simulink model "srmc_sensor_controller_model"  (R2025a)
settings: Solver=FixedStepDiscrete  StartTime=0.0  StopTime=86400  FixedStep=300  RelTol=1e-3
settings Model: Creator=ELCOT  LastModifiedBy=ELCOT

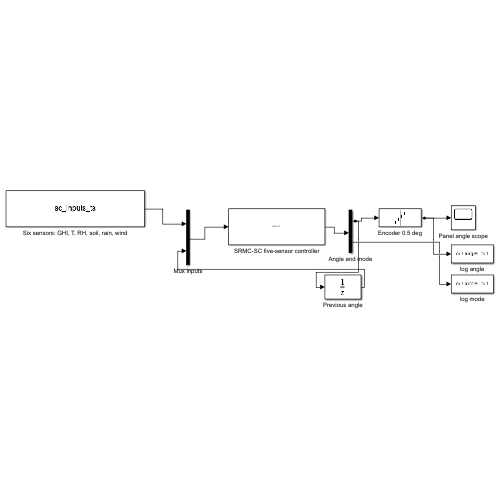
[thumbnail: Simulink's stored preview of the top-level diagram]
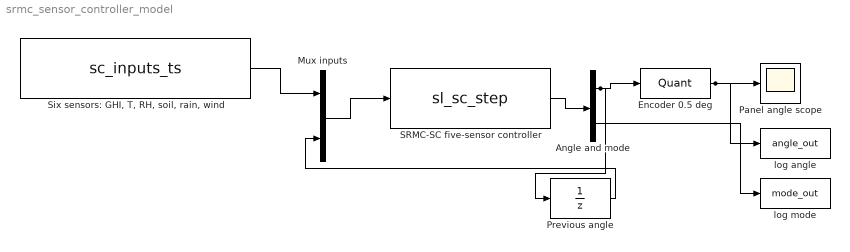
== system srmc_sensor_controller_model ==
  Angle and mode : Demux  Outputs=2
  Encoder 0.5 deg : Quantizer
  Mux inputs : Mux  Inputs=2
  Panel angle scope : Scope
  Previous angle : UnitDelay  InitialCondition=15  SampleTime=300  HasFrameUpgradeWarning=on
  SRMC-SC five-sensor controller : MATLABFcn  MATLABFcn=sl_sc_step  OutputDimensions=2
  "Six sensors: GHI, T, RH, soil, rain, wind" : FromWorkspace  VariableName=sc_inputs_ts  SampleTime=300
  log angle : ToWorkspace  VariableName=angle_out  SampleTime=-1
  log mode : ToWorkspace  VariableName=mode_out  SampleTime=-1
  wires:
  "Six sensors: GHI, T, RH, soil, rain, wind"/1 -> Mux inputs/1
  Previous angle/1 -> Mux inputs/2
  Mux inputs/1 -> SRMC-SC five-sensor controller/1
  SRMC-SC five-sensor controller/1 -> Angle and mode/1
  Angle and mode/1 -> Encoder 0.5 deg/1, Previous angle/1
  Encoder 0.5 deg/1 -> Panel angle scope/1, log angle/1
  Angle and mode/2 -> log mode/1
